simulink model "dsPIC_32MX360F512L_Proba"  (Simulink 7.3)
settings: Solver=FixedStepDiscrete  StartTime=0.0  StopTime=10  FixedStep=0.5  RelTol=1e-3
undefined symbols (not defined in the file or in its folder): configSPI, sendSPI, setport, u1
libraries: dsPICdrivers x6
settings Model: Creator=Lubin  LastModifiedBy=Matija
settings OptimizationCC: InlineParams=on  InlineInvariantSignals=on  EnforceIntegerDowncast=off  StateBitsets=on  DataBitsets=on  UseTempVars=on  ZeroExternalMemoryAtStartup=off  ZeroInternalMemoryAtStartup=off  OptimizeModelRefInitCode=on  LifeSpan=1
settings DebuggingCC: SaveWithParameterizedLinksMsg=none  SignalResolutionControl=TryResolveAllWithWarning
settings HardwareCC: TargetHWDeviceType=32-bit Generic
settings RTWCC: SystemTargetFile=pic32.tlc  TemplateMakefile=pic32_gcc.tmf  PostCodeGenCommand=dsPIC_Compile()  Description=Embedded Target for Microchip dsPIC (real-time)  ProcessScript=pic32_make_rtw_hook  CustomSource=Function.c
settings CodeAppCC: IgnoreCustomStorageClasses=off
settings STFCustomTargetCC: TargetFcnLib=ansi_tfl_tmw.mat  ModelReferenceCompliant=off  IncludeMdlTerminateFcn=off  CombineOutputUpdateFcns=on  SuppressErrorStatus=on  ERTCustomFileBanners=on  SupportContinuousTime=off  SupportNonInlinedSFcns=off  CPPClassGenCompliant=on  SystemTargetFile=pic32.tlc
settings ERTTargetCC: TargetFcnLib=ansi_tfl_tmw.mat  MultiwordLength=2048  ModelReferenceCompliant=off  ParMdlRefBuildCompliant=off  CompOptLevelCompliant=off  IncludeMdlTerminateFcn=off  SuppressErrorStatus=on  ERTFirstTimeCompliant=off  ModelStepFunctionPrototypeControlCompliant=off  ExtModeMexFile=noextcomm  InlinedParameterPlacement=NonHierarchical  ERTSrcFileBannerTemplate=dsPIC_code_template.cgt  ERTHdrFileBannerTemplate=dsPIC_code_template.cgt  ERTDataSrcFileTemplate=dsPIC_code_template.cgt  ERTDataHdrFileTemplate=dsPIC_code_template.cgt  ERTCustomFileTemplate=dsPIC_main.tlc
settings CustomProperty: DataType=string  Value=C:\PROGRA~1\MATLAB\R2009a\bin\win32\gmake

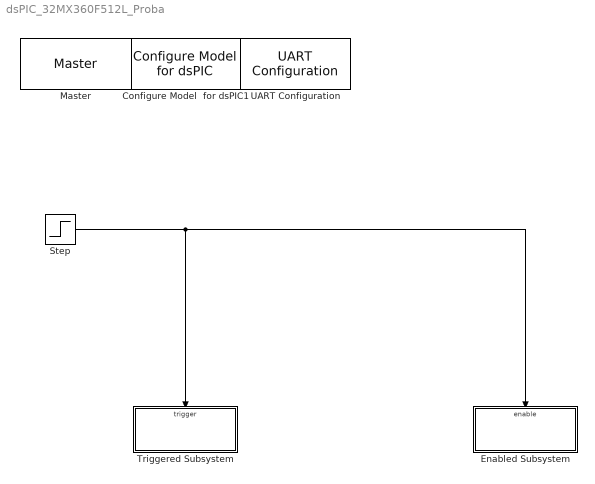
== system dsPIC_32MX360F512L_Proba ==
  Configure Model  for dsPIC1 : dsPICdrivers/Simulink Configuration/Configure Model  for dsPIC
  Enabled Subsystem : Subsystem  TreatAsAtomicUnit=on
  Master : dsPICdrivers/Master  Tag=dsPIC_MASTER  Priority=1  TimeStepType=Timer1  picType=32MX360F512L  fcy=16000000  Quartz_33f=8e6  PLLActive_33f=on  fcyDesired_33f=16e6  tmr1="[256  31249  0]"  tmr1Info="Time Step : 0.5  ;   Error : 0%  PR1=31249"  tmr2345="[0  0  0  0]"  tmr2345cfg=[-1 -1 -1 -1]  IOautoConf=on  typePort="[ 0  0  0  0  0  0  0  0  0  0  0  0  0  0  0  0  0  0  0  0  0  0  0  0  0  0  0  0  0  0  0  0  0  0  0  0  0  0  0  0  0  0  0  0  0  0  0  0  0  0  0  0  0  0  0  0  0  0  0  0  0  0  0  0  0  0  0  0  0  0  0  0  0  0  0  0  0  0  0  0  0  0  4  0  0  0  0  0  0  0  0  0  0  0  0  0  0  0  0  0  0  0  0  0  0  0  0  0  0  0  0  0 ]"  TRIS="[ 65535  65535  65535  65535  65535  65535  65535 ]"  ADPCFG=0  MasterBusyPort=None  MasterOverloadPort=None  FOSC=Quartz (XT - HS)  ClockSwitchMonitor=Both disabled  TempProtection_33f=TEMP_ON  FPBOR=<empty>  PWRT=disable  MCLR=<empty>  ICD=ICS_NONE  JTAGEN=JTAGEN_OFF  PowerSave=off  OverrideFcy=off  NewFcy=1e6  PR2345="[65535  65535  65535  65535]"
  Step : Step  Time=0.5
  Triggered Subsystem : Subsystem  TreatAsAtomicUnit=on
  UART Configuration : dsPICdrivers/Serial PORT/UART Configuration  Tag=dsPIC_config_UART  Priority=2  UART=1  proposed_BAUD=115200  ALT_TX_RX=on  InterruptTxWhen=When Transmit Buffer is empty  TXInterruptPri=1  TxBufferSize=32  TXEN=off  InterruptRxWhen=When a character is received  RXInterruptPri=6  RxBufferSize=32  BAUD=115200  UxBRG=8  Info="UxBRG = 8   ||  Real Baud : 111111   ||  % error : -3.5494  ||  max 5555.5556 Bytes / Step"  RealBaud=0
  wires:
  Step/1 -> Triggered Subsystem/Trigger, Enabled Subsystem/Enable

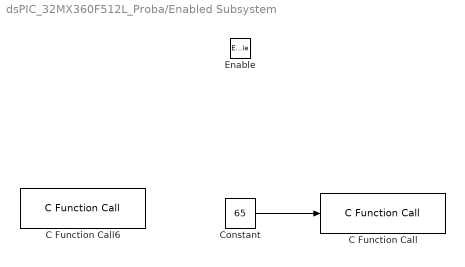
== system dsPIC_32MX360F512L_Proba/Enabled Subsystem ==
  Enable : EnablePort
  C Function Call : dsPICdrivers/OTHERS/C Function Call  Tag=dsPIC_dsPIC_CFunctionCall  fctName='sendSPI'  INPUT_SIZE=1  INPUT1=int8  INPUT2=--  INPUT3=--  OUTPUT_SIZE=1  OUTPUT1=--  SampleTime=-1  InputType=[ 1 ]  OutputType=[ ]  FctDeclaration=extern void sendSPI(int8_T u1);  FctCall=sendSPI(%u1);  OrderingInOutPopup=None
  C Function Call6 : dsPICdrivers/OTHERS/C Function Call  Tag=dsPIC_dsPIC_CFunctionCall  fctName='setport'  INPUT_SIZE=1  INPUT1=--  INPUT2=--  INPUT3=--  OUTPUT_SIZE=1  OUTPUT1=--  SampleTime=-1  InputType=[ ]  OutputType=[ ]  FctDeclaration=extern void setport();  FctCall=setport();  OrderingInOutPopup=None
  Constant : Constant  Value=65  OutDataTypeMode=int8  OutDataType=fixdt(1, 16)  OutScaling=2^0  OutDataTypeStr=int8  SampleTime=-1
  wires:
  Constant/1 -> C Function Call/1

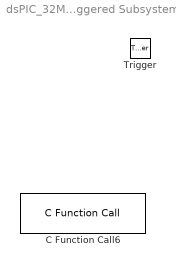
== system dsPIC_32MX360F512L_Proba/Triggered Subsystem ==
  Trigger : TriggerPort
  C Function Call6 : dsPICdrivers/OTHERS/C Function Call  Tag=dsPIC_dsPIC_CFunctionCall  fctName='configSPI'  INPUT_SIZE=1  INPUT1=--  INPUT2=--  INPUT3=--  OUTPUT_SIZE=1  OUTPUT1=--  SampleTime=-1  InputType=[ ]  OutputType=[ ]  FctDeclaration=extern void configSPI();  FctCall=configSPI();  OrderingInOutPopup=None
